simulink model "TeresaP5NP"  (R2023b)
settings: Solver=VariableStepAuto  StartTime=0.0  StopTime=450  RelTol=1e-3
settings Model: Creator=34697  LastModifiedBy=34697

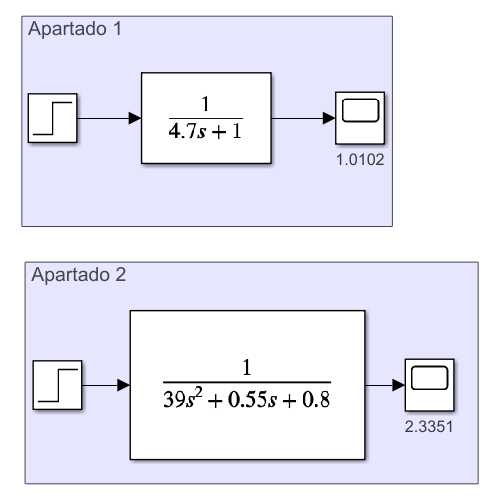
[thumbnail: Simulink's stored preview of the top-level diagram]
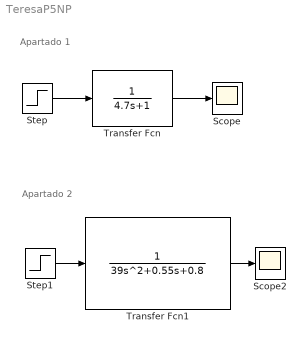
== system TeresaP5NP ==
  note: Apartado 2
  note: Apartado 1
  Scope : Scope
      settings: AttributesFormatString=%<ActiveDisplayYMaximum>
  Scope2 : Scope
      settings: AttributesFormatString=%<ActiveDisplayYMaximum>
  Step : Step  SampleTime=0
  Step1 : Step  SampleTime=0
  Transfer Fcn : TransferFcn  Denominator=[4.7 1]
  Transfer Fcn1 : TransferFcn  Denominator=[39 0.55 0.8]
  wires:
  Transfer Fcn/1 -> Scope/1
  Step/1 -> Transfer Fcn/1
  Transfer Fcn1/1 -> Scope2/1
  Step1/1 -> Transfer Fcn1/1
